simulink model "Touchdown_Stop"  (R2026b)
settings: Solver=VariableStepAuto
libraries: simulink x1
settings Model: Creator=asing  LastModifiedBy=David

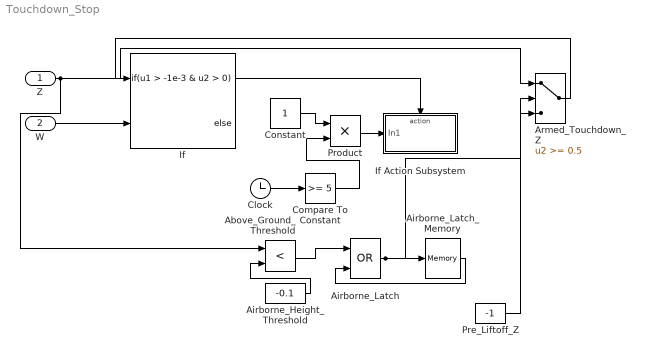
== system Touchdown_Stop ==
  Z : Inport
  W : Inport  Port=2
  Above_Ground_Threshold : RelationalOperator  Operator=<  OutDataTypeStr=boolean  RndMeth=Simplest  InputSameDT=off
  Airborne_Height_Threshold : Constant  Value=-0.1
  Airborne_Latch : Logic  Operator=OR  AllPortsSameDT=off  OutDataTypeStr=boolean
  Airborne_Latch_Memory : Memory
  Armed_Touchdown_Z : Switch  Threshold=0.5  SaturateOnIntegerOverflow=off  InputSameDT=off
  Clock : Clock
  Compare To Constant : simulink/Logic and Bit Operations/Compare To Constant  relop=>=  const=5  OutDataTypeStr=boolean
  Constant : Constant
  If : If  NumInputs=2  IfExpression=u1 > -1e-3 & u2 > 0
  If Action Subsystem : Subsystem  TreatAsAtomicUnit=on
  Pre_Liftoff_Z : Constant  Value=-1
  Product : Product
  wires:
  W/1 -> If/2
  If/1 -> If Action Subsystem/Action
  Clock/1 -> Compare To Constant/1
  Compare To Constant/1 -> Product/2
  Constant/1 -> Product/1
  Product/1 -> If Action Subsystem/1(In1)
  Z/1 -> Above_Ground_Threshold/1, Armed_Touchdown_Z/1
  Airborne_Height_Threshold/1 -> Above_Ground_Threshold/2
  Above_Ground_Threshold/1 -> Airborne_Latch/1
  Airborne_Latch_Memory/1 -> Airborne_Latch/2
  Airborne_Latch/1 -> Airborne_Latch_Memory/1, Armed_Touchdown_Z/2
  Pre_Liftoff_Z/1 -> Armed_Touchdown_Z/3
  Armed_Touchdown_Z/1 -> If/1

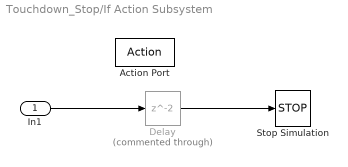
== system Touchdown_Stop/If Action Subsystem ==
  In1 : Inport
  Action Port : ActionPort
  Delay : Delay  Commented=through
  Stop Simulation : Stop
  wires:
  Delay/1 -> Stop Simulation/1
  In1/1 -> Delay/1
